simulink model "Cognitive_Radio_Model_backup_final"  (R2023a)
settings: Solver=VariableStepAuto  StartTime=0.0  StopTime=30.0  RelTol=1e-3
libraries: simulink x2
settings Model: Creator=Deepak1  LastModifiedBy=Deepak1

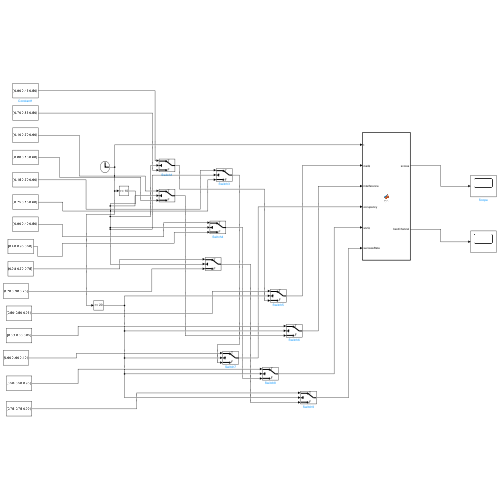
[thumbnail: Simulink's stored preview of the top-level diagram]
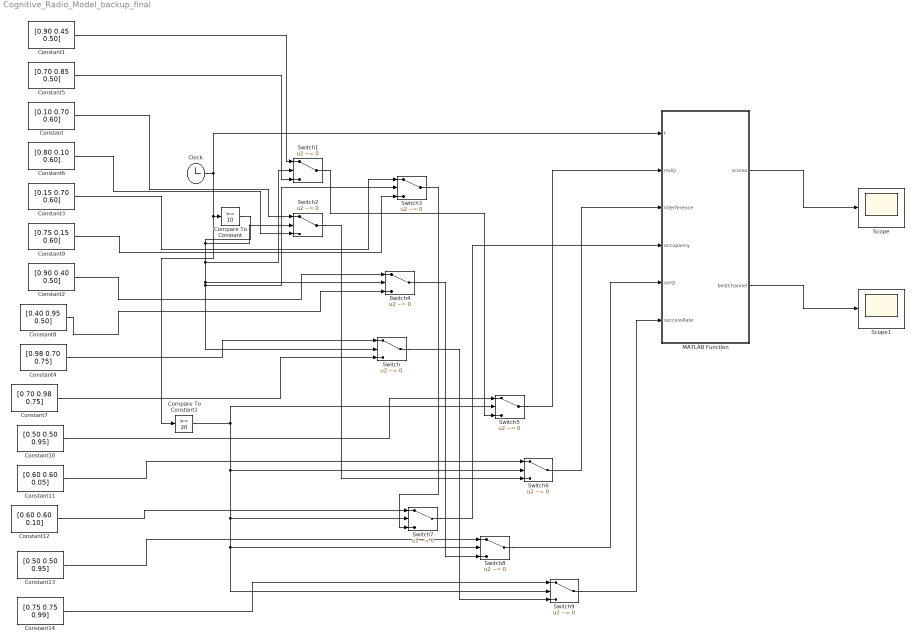
== system Cognitive_Radio_Model_backup_final ==
  Clock : Clock
  Compare To Constant : simulink/Logic and Bit Operations/Compare To Constant  relop=>=  const=10  OutDataTypeStr=boolean
  Compare To Constant1 : simulink/Logic and Bit Operations/Compare To Constant  relop=>=  const=20  OutDataTypeStr=boolean
  Constant : Constant  Value=[0.10 0.70 0.60]
  Constant1 : Constant  Value=[0.90 0.45 0.50]
  Constant10 : Constant  Value=[0.50 0.50 0.95]
  Constant11 : Constant  Value=[0.60 0.60 0.05]
  Constant12 : Constant  Value=[0.60 0.60 0.10]
  Constant13 : Constant  Value=[0.50 0.50 0.95]
  Constant14 : Constant  Value=[0.75 0.75 0.99]
  Constant2 : Constant  Value=[0.90 0.40 0.50]
  Constant3 : Constant  Value=[0.15 0.70 0.60]
  Constant4 : Constant  Value=[0.98 0.70 0.75]
  Constant5 : Constant  Value=[0.70 0.85 0.50]
  Constant6 : Constant  Value=[0.80 0.10 0.60]
  Constant7 : Constant  Value=[0.70 0.98 0.75]
  Constant8 : Constant  Value=[0.40 0.95 0.50]
  Constant9 : Constant  Value=[0.75 0.15 0.60]
  MATLAB Function : MATLAB Function  TreatAsAtomicUnit=on
  Scope : Scope
  Scope1 : Scope
  Switch{,1..9} (10 alike) : Switch  Criteria=u2 ~= 0  SaturateOnIntegerOverflow=off  InputSameDT=off
  wires:
  MATLAB Function/1(scores) -> Scope/1
  MATLAB Function/2(bestChannel) -> Scope1/1
  Clock/1 -> Compare To Constant1/1, Compare To Constant/1, MATLAB Function/1(t)
  Compare To Constant/1 -> Switch/2, Switch3/2, Switch4/2, Switch1/2, Switch2/2
  Constant5/1 -> Switch1/3
  Switch1/1 -> Switch5/3
  Constant1/1 -> Switch1/1
  Constant/1 -> Switch2/1
  Constant6/1 -> Switch2/3
  Switch2/1 -> Switch6/3
  Constant3/1 -> Switch3/1
  Constant9/1 -> Switch3/3
  Switch3/1 -> Switch7/3
  Constant2/1 -> Switch4/1
  Constant8/1 -> Switch4/3
  Switch/1 -> Switch9/3
  Constant4/1 -> Switch/1
  Constant7/1 -> Switch/3
  Switch4/1 -> Switch8/3
  Compare To Constant1/1 -> Switch9/2, Switch8/2, Switch7/2, Switch6/2, Switch5/2
  Constant10/1 -> Switch5/1
  Constant11/1 -> Switch6/1
  Constant12/1 -> Switch7/1
  Constant13/1 -> Switch8/1
  Constant14/1 -> Switch9/1
  Switch9/1 -> MATLAB Function/6(successRate)
  Switch8/1 -> MATLAB Function/5(snrQ)
  Switch7/1 -> MATLAB Function/4(occupancy)
  Switch6/1 -> MATLAB Function/3(interference)
  Switch5/1 -> MATLAB Function/2(rssiQ)

== matlab function Cognitive_Radio_Model_backup_final/MATLAB Function ==
  data: t input; scores output; bestChannel output; rssiQ input; interference input; occupancy input; snrQ input; successRate input
function [scores, bestChannel] = fcn(t, rssiQ, interference, occupancy, snrQ, successRate)

baseScores = 0.20 .* rssiQ ...
           + 0.25 .* (1 - interference) ...
           + 0.20 .* (1 - occupancy) ...
           + 0.20 .* snrQ ...
           + 0.15 .* successRate;

if t < 10
    preferredIdx = 1;
elseif t < 20
    preferredIdx = 2;
else
    preferredIdx = 3;
end

scores = baseScores;
scores(preferredIdx) = max(baseScores) + 0.01;
scores = scores ./ max(scores);

[~, idx] = max(scores);
channels = [1 6 11];
bestChannel = channels(idx);

end
